simulink model "SMC_AEM"  (R2026b)
settings Model: Creator=Yahoff  LastModifiedBy=Yahoff

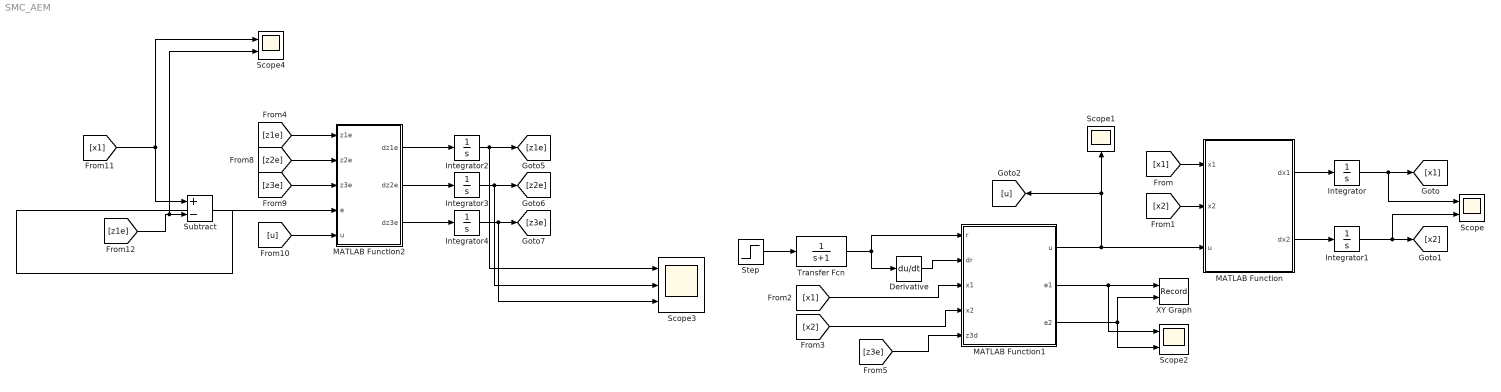
== system SMC_AEM ==
  Derivative : Derivative
  Integrator : Integrator  InitialCondition=-2
  Integrator1 : Integrator  InitialCondition=-2
  Integrator2 : Integrator
  Integrator3 : Integrator
  Integrator4 : Integrator
  MATLAB Function : MATLAB Function  TreatAsAtomicUnit=on
  MATLAB Function1 : MATLAB Function  TreatAsAtomicUnit=on
  MATLAB Function2 : MATLAB Function  TreatAsAtomicUnit=on
  Scope : Scope  NumInputPorts=2
      settings: ActiveDisplayYMinimum=-3.4521381362399395  ActiveDisplayYMaximum=4.7296149016922016
  Scope1 : Scope
      settings: ActiveDisplayYMinimum=-25.367974300020894  ActiveDisplayYMaximum=46.905143277646424
  Scope2 : Scope  NumInputPorts=2
      settings: ActiveDisplayYMinimum=-0.67609996049472021  ActiveDisplayYMaximum=2.3743732511818694  DataLoggingVariableName=ScopeData2
  Scope3 : Scope  NumInputPorts=3
      settings: ActiveDisplayYMinimum=-2.4943647722506022  ActiveDisplayYMaximum=1.7379857549794822  DataLoggingVariableName=ScopeData3
  Scope4 : Scope  NumInputPorts=2
      settings: ActiveDisplayYMinimum=-2.6687109642083282  ActiveDisplayYMaximum=3.19643954119239  DataLoggingVariableName=ScopeData4
  Step : Step  SampleTime=0
  Subtract : Sum  Inputs=+-
  Transfer Fcn : TransferFcn  Denominator=[1 1]
  XY Graph : Record  NumPorts=2.0  FileSettingsInternal="{\"entries\":[{\"content\":{\"excelSettings\":{\"content\":{},\"type\":\"Streamout.ExcelSettings\"},\"parquetSettings\":{\"content\":{},\"type\":\"Streamout.ParquetSettings\"}},\"type\":\"Streamout.FileSettingStorage\",\"uuid\":\"\"}],\"packageUris\":[\"http:\\/\\/schema.mathworks.com\\/mf0\\/streamout_blocks\\/R2020a\"],\"version\":\"1.0\"}"  FrameSettings=[0, 0]  Layout=[1 1]  SignalsInternal="{\"entries\":[{\"content\":{\"signals\":[{\"content\":{\"blockPath\":[],\"dimensions\":[1],\"domain\":\"\",\"lineColor\":\"#a2142f\",\"lineWidth\":2,\"port\":1,\"sid\":[\"\"],\"signalID\":1,\"signalName\":\"MATLAB Function1:2\"},\"type\":\"RecordBlkView.Signal\",\"uuid\":\"\"},{\"content\":{\"blockPath\":[],\"dimensions\":[1],\"domain\":\"\",\"lineColor\":\"#139fff\",\"lineWidth\":2,\"port\":2,\"sid\":[\"\"],\"signalID\":2,\"signalName\":\"MATLAB Function1:3\"},\"type\":\"RecordBlkView.Signal\",\"uuid\":\"\"}]},\"type\":\"RecordBlkView.InputSignals\",\"uuid\":\"\"}],\"packageUris\":[\"http:\\/\\/schema.mathworks.com\\/mf0\\/streamout_blocks\\/R2020a\"],\"version\":\"1.0\"}"  VisualizationBindings="{\"xyplotplugin\":{\"info\":[{\"series\":[{\"bindingParametersList\":[{\"parameter\":\"X-Axis\",\"signalID\":6326,\"signalName\":\"MATLAB Function1:2\"},{\"parameter\":\"Y-Axis\",\"signalID\":6330,\"signalName\":\"MATLAB Function1:3\"}],\"seriesID\":0}],\"subplotID\":1}]}}"  CompatibilityTag=XY
  wires:
  MATLAB Function/1(dx1) -> Integrator/1
  MATLAB Function/2(dx2) -> Integrator1/1
  Integrator/1 -> Scope/1, [x1]
  Integrator1/1 -> Scope/2, [x2]
  [x1] -> MATLAB Function/1(x1)
  [x2] -> MATLAB Function/2(x2)
  MATLAB Function1/1(u) -> MATLAB Function/3(u), [u], Scope1/1
  Derivative/1 -> MATLAB Function1/2(dr)
  [x1] -> MATLAB Function1/3(x1)
  [x2] -> MATLAB Function1/4(x2)
  MATLAB Function1/2(e1) -> Scope2/1, XY Graph/1
  MATLAB Function1/3(e2) -> Scope2/2, XY Graph/2
  MATLAB Function2/2(dz2e) -> Integrator3/1
  [u] -> MATLAB Function2/5(u)
  [z1e] -> Scope4/2, Subtract/2
  [z1e] -> MATLAB Function2/1(z1e)
  Integrator2/1 -> Scope3/1, [z1e]
  Subtract/1 -> MATLAB Function2/4(e)
  [x1] -> Subtract/1, Scope4/1
  Integrator3/1 -> Scope3/2, [z2e]
  [z2e] -> MATLAB Function2/2(z2e)
  MATLAB Function2/1(dz1e) -> Integrator2/1
  [z3e] -> MATLAB Function2/3(z3e)
  Integrator4/1 -> Scope3/3, [z3e]
  MATLAB Function2/3(dz3e) -> Integrator4/1
  Step/1 -> Transfer Fcn/1
  Transfer Fcn/1 -> MATLAB Function1/1(r), Derivative/1
  [z3e] -> MATLAB Function1/5(z3d)

== matlab function SMC_AEM/MATLAB Function1 ==
  data: r input; u output; dr input; x1 input; x2 input; e1 output; e2 output; z3d input
function [u,e1,e2] = fcn(r,dr,x1,x2,z3d)

m = 2;
K = 1;

%z3d=0;

e1 = r - x1;
e2 = dr - x2;

s = e2 + m*e1;

u = -z3d + m*e2 + K*sign(s);

== matlab function SMC_AEM/MATLAB Function ==
  data: x1 input; x2 input; u input; dx1 output; dx2 output
function [dx1,dx2] = fcn(x1,x2,u)

dx1 = sin(x1+x2)+x2;
dx2 = cos(x1+x2)+u;

== matlab function SMC_AEM/MATLAB Function2 ==
  data: z1e input; z2e input; z3e input; e input; u input; dz1e output; dz2e output; dz3e output
function [dz1e,dz2e,dz3e] = fcn(z1e,z2e,z3e,e,u)

b=1;
K1=0.459e+3;     %6
K2=1.1562e+3;    %21
K3=8.6543e+3;    %23

dz1e = z2e + K1*e;

dz2e = z3e + b*u + K2*e;

dz3e = K3*e;
